simulink model "bouncing_ball_R2018a"  (R2018a)
settings: Solver=FixedStepDiscrete  StartTime=0.0  StopTime=25  FixedStep=Ts  MaxStep=1e-3  RelTol=1e-3
values from neighbouring files (symbols this model uses):
  coefficient_of_restitution = Simulink.Parameter    [bouncing_ball_benchmark.m]    (also in bouncing_ball_init.m)
  gravitational_constant = Simulink.Parameter    [bouncing_ball_benchmark.m]    (also in bouncing_ball_init.m)
undefined symbols (not defined in the file or in its folder): DiscIntNeverNeededParam
libraries: simulink x1
settings Model: Creator=user  LastModifiedBy=admin
settings OptimizationCC: DefaultParameterBehavior=Inlined  EnhancedBackFolding=on  PassReuseOutputArgsAs=Individual arguments  OptimizeBlockOrder=speed  DifferentSizesBufferReuse=on  OptimizationCustomize=off
settings DebuggingCC: ParameterTunabilityLossMsg=error
settings HardwareCC: TargetBitPerPointer=64  TargetBitPerSizeT=64  TargetBitPerPtrDiffT=64  TargetLongLongMode=on  TargetIntDivRoundTo=Zero  TargetEndianess=LittleEndian  TargetWordSize=64  TargetHWDeviceType=MATLAB Host  ProdEqTarget=off
settings SFSimCC: SimUseLocalCustomCode=on  MATLABDynamicMemAlloc=off
settings RTWCC: Description=Embedded Coder (host-based shared library target)  SystemTargetFile=ert_shrlib.tlc  TemplateMakefile=ert_default_tmf  GenerateReport=on  RTWUseLocalCustomCode=on  BuildConfiguration=Faster Runs  IncludeHyperlinkInReport=on  LaunchReport=on  GenerateTraceInfo=on  GenerateTraceReport=on  GenerateTraceReportSl=on  GenerateTraceReportSf=on  GenerateTraceReportEml=on
settings CodeAppCC: ForceParamTrailComments=on  IgnoreCustomStorageClasses=off  OperatorAnnotations=on  SimulinkDataObjDesc=on  SFDataObjDesc=on  InsertBlockDesc=on
settings STFCustomTargetCC: TargetLangStandard=C99 (ISO)  MultiwordLength=256  GenerateSampleERTMain=on  ParMdlRefBuildCompliant=on  CompOptLevelCompliant=on  CombineOutputUpdateFcns=on  ERTCustomFileBanners=on  SupportContinuousTime=off  SupportNonInlinedSFcns=off  RemoveResetFunc=on  MATLABClassNameForMDSCustomization=Simulink.SoftwareTarget.ERTCustomization  ModelStepFunctionPrototypeControlCompliant=on  GRTInterface=off  UseToolchainInfoCompliant=on  SystemTargetFile=ert_shrlib.tlc
settings ERTTargetCC: TargetLangStandard=C99 (ISO)  GenerateSampleERTMain=on  ConcurrentExecutionCompliant=off  CPPClassGenCompliant=off  InlinedParameterPlacement=NonHierarchical  ERTCustomFileTemplate=example_file_process.tlc

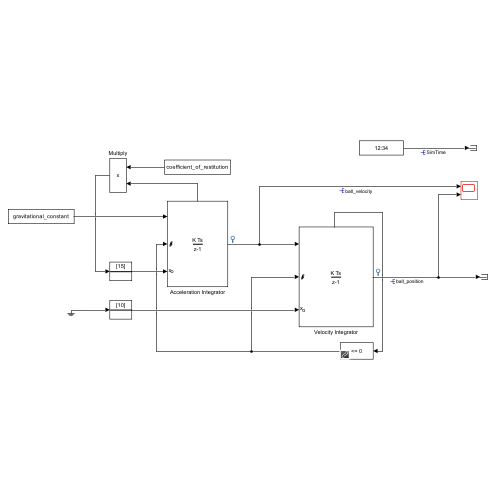
[thumbnail: Simulink's stored preview of the top-level diagram]
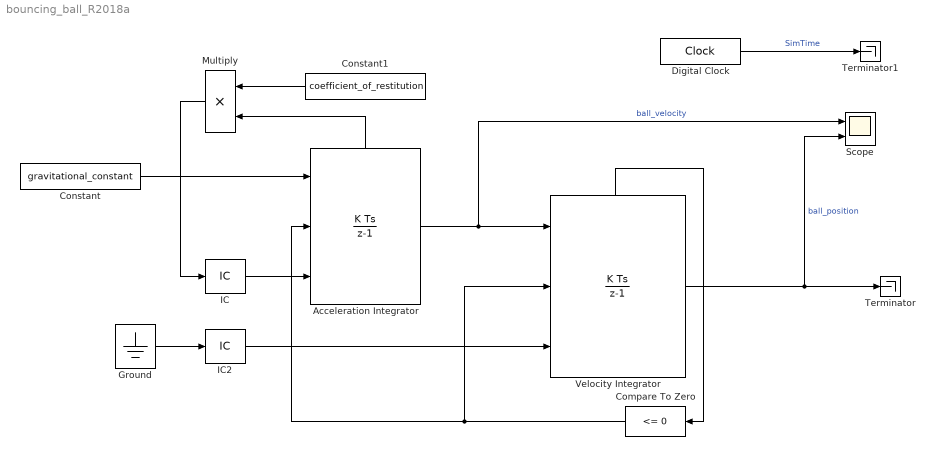
== system bouncing_ball_R2018a ==
  Acceleration Integrator : DiscreteIntegrator  ExternalReset=rising  InitialConditionSource=external  SampleTime=-1  OutDataTypeStr=single  ShowStatePort=on  ICPrevOutput=DiscIntNeverNeededParam  ICPrevScaledInput=DiscIntNeverNeededParam
  Compare To Zero : simulink/Logic and Bit Operations/Compare To Zero  relop=<=  OutDataTypeStr=boolean
  Constant : Constant  Value=gravitational_constant  OutMin=-25  OutMax=25  OutDataTypeStr=single
  Constant1 : Constant  Value=coefficient_of_restitution  OutDataTypeStr=single
  Digital Clock : DigitalClock  SampleTime=1e-3
  Ground : Ground
  IC : InitialCondition  Value=15
  IC2 : InitialCondition  Value=10
  Multiply : Product  OutDataTypeStr=Inherit: Same as first input
  Scope : Scope  NumInputPorts=2
  Terminator : Terminator
  Terminator1 : Terminator
  Velocity Integrator : DiscreteIntegrator  ExternalReset=rising  InitialConditionSource=external  SampleTime=-1  ShowStatePort=on  ICPrevOutput=DiscIntNeverNeededParam  ICPrevScaledInput=DiscIntNeverNeededParam
  wires:
  Constant/1 -> Acceleration Integrator/1
  IC/1 -> Acceleration Integrator/3
  Acceleration Integrator/State -> Multiply/2
  Ground/1 -> IC2/1
  Acceleration Integrator/1 -> Scope/1, Velocity Integrator/1  "ball_velocity"
  IC2/1 -> Velocity Integrator/3
  Compare To Zero/1 -> Velocity Integrator/2, Acceleration Integrator/2
  Velocity Integrator/State -> Compare To Zero/1
  Velocity Integrator/1 -> Scope/2, Terminator/1  "ball_position"
  Multiply/1 -> IC/1
  Constant1/1 -> Multiply/1
  Digital Clock/1 -> Terminator1/1  "SimTime"
